simulink model "linear_analysis_model"  (R2024b)
settings: Solver=ode4  StartTime=0.0  StopTime=40  FixedStep=0.001  RelTol=1e-3
PreLoadFcn:
  | run('JacobianAnalysis.m')
InitFcn:
  | run('JacobianAnalysis.m')
values from neighbouring files (symbols this model uses):
  A_analysis = double(A_analysis)    [JacobianAnalysis.m]
  B_analysis = double(B_analysis)    [JacobianAnalysis.m]
  X0 = [op_trim3.States(1, 1).x;op_trim3.States(2,1).x;op_trim3.States(3,1).x;op_trim3.States(4,1).x]    [JacobianAnalysis.m]
undefined symbols (not defined in the file or in its folder): op_trim3
settings Model: Creator=LocoalKOH  LastModifiedBy=LocoalKOH

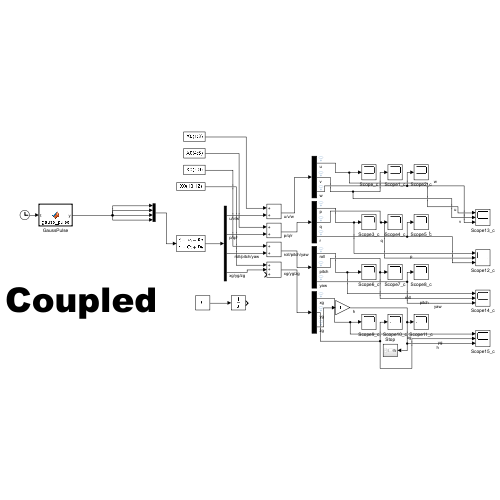
[thumbnail: Simulink's stored preview of the top-level diagram]
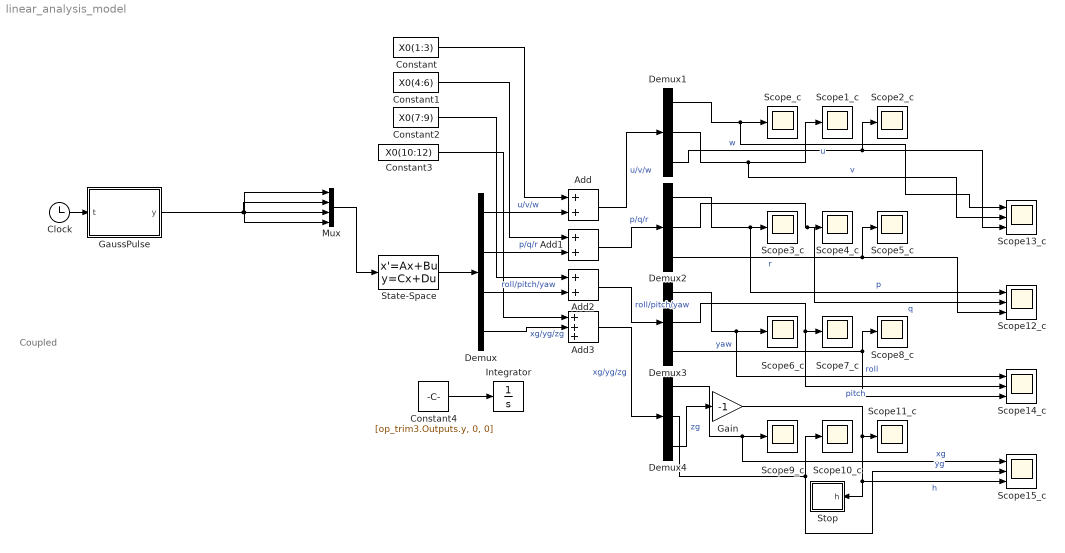
== system linear_analysis_model ==
  note: Coupled
  Add : Sum
  Add1 : Sum
  Add2 : Sum
  Add3 : Sum  Inputs=+++
  Clock : Clock
  Constant : Constant  Value=X0(1:3)  VectorParams1D=off
  Constant1 : Constant  Value=X0(4:6)  VectorParams1D=off
  Constant2 : Constant  Value=X0(7:9)  VectorParams1D=off
  Constant3 : Constant  Value=X0(10:12)  VectorParams1D=off
  Constant4 : Constant  Value=[op_trim3.Outputs.y, 0, 0]
  Demux : Demux
  Demux{1..4} (4 alike) : Demux  Outputs=3
  Gain : Gain  Gain=-1
  GaussPulse : MATLAB Function  TreatAsAtomicUnit=on
  Integrator : Integrator
  Mux : Mux
  Scope10_c : Scope
  Scope11_c : Scope
  Scope12_c : Scope  NumInputPorts=3
  Scope13_c : Scope  NumInputPorts=3
  Scope14_c : Scope  NumInputPorts=3
  Scope15_c : Scope  NumInputPorts=3
  Scope1_c : Scope
  Scope2_c : Scope
  Scope3_c : Scope
  Scope4_c : Scope
  Scope5_c : Scope
  Scope6_c : Scope
  Scope7_c : Scope
  Scope8_c : Scope
  Scope9_c : Scope
  Scope_c : Scope
  State-Space : StateSpace  A=A_analysis  B=B_analysis  C=eye(12)  D=zeros(12,4)  InitialCondition=zeros(12,1)  ContinuousStateAttributes={'u','v','w','p','q','r','roll','pitch','yaw','xg','yg','zg'}
  Stop : Subsystem
  wires:
  Constant3/1 -> Add3/1
  State-Space/1 -> Demux/1
  Demux/4 -> Add3/2  "xg/yg/zg"
  Demux/3 -> Add2/2  "roll/pitch/yaw"
  Constant2/1 -> Add2/1
  Constant/1 -> Add/1
  Demux/2 -> Add1/2  "p/q/r"
  Constant1/1 -> Add1/1
  Demux/1 -> Add/2  "u/v/w"
  Mux/1 -> State-Space/1
  Constant4/1 -> Integrator/1
  Demux4/1 -> Scope15_c/1, Scope9_c/1  "xg"
  Demux1/3 -> Scope13_c/3, Scope2_c/1  "w"
  Demux3/2 -> Scope14_c/2, Scope7_c/1  "pitch"
  Demux1/2 -> Scope13_c/2, Scope1_c/1  "v"
  Demux4/3 -> Gain/1  "zg"
  Demux3/3 -> Scope14_c/3, Scope8_c/1  "yaw"
  Demux1/1 -> Scope13_c/1, Scope_c/1  "u"
  Demux3/1 -> Scope14_c/1, Scope6_c/1  "roll"
  Demux2/1 -> Scope12_c/1, Scope3_c/1  "p"
  Gain/1 -> Scope11_c/1, Scope15_c/3, Stop/1(h)  "h"
  Demux2/2 -> Scope12_c/2, Scope4_c/1  "q"
  Demux2/3 -> Scope12_c/3, Scope5_c/1  "r"
  Demux4/2 -> Scope15_c/2, Scope10_c/1  "yg"
  Add/1 -> Demux1/1  "u/v/w"
  Add1/1 -> Demux2/1  "p/q/r"
  Add2/1 -> Demux3/1  "roll/pitch/yaw"
  Add3/1 -> Demux4/1  "xg/yg/zg"
  Clock/1 -> GaussPulse/1(t)
  GaussPulse/1(y) -> Mux/4, Mux/3, Mux/1, Mux/2

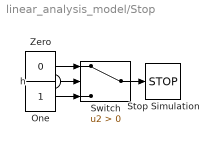
== system linear_analysis_model/Stop ==
  h : Inport
  One : Constant  OutDataTypeStr=Inherit: Inherit via back propagation
  Stop Simulation : Stop
  Switch : Switch  Criteria=u2 > Threshold  SaturateOnIntegerOverflow=off  InputSameDT=off
  Zero : Constant  Value=0  OutDataTypeStr=Inherit: Inherit via back propagation
  wires:
  One/1 -> Switch/3
  Zero/1 -> Switch/1
  Switch/1 -> Stop Simulation/1
  h/1 -> Switch/2

== matlab function linear_analysis_model/GaussPulse ==
  data: t input; y output
function y = gauss_pulse(t)
    y = 0.1 * exp(-(t - 5)^2 / 0.1);  % 在t=5秒附近有扰动
end
